simulink model "ASM_Traffic"  (R2026a)
settings: Solver=ode1  StartTime=SIM.tstart.v  StopTime=SIM.tend.v  FixedStep=SIM.StepSize.v
PostLoadFcn:
  | if any(exist('dsrtsu_mdlpostloadfcn', 'file') ~= 0), dsrtsu_mdlpostloadfcn('Execute', bdroot); end
  | try, asm_mdl_postloadfcn(bdroot, 'UpdateModel', 3600); catch, disp(lasterr); end,
InitFcn:
  | , if any(exist('rtifpga_mdlclblib', 'file') ~= 0), rtifpga_mdlclblib('Init', bdroot); end,
  | , if any(exist('dsmpb_private', 'file') ~= 0), dsmpb_private('dsmpb_mdlclblib', 'Init', bdroot); end,
model workspace (MAT data in the model file):
  asmReferencePath = [0 0.01 0.02 0.03 0.04 0.05 0.06 0.07 0.08 0.09 0.1 0.11 ... (350007 elements, 50001x7)]
  roadBounds : Simulink.Parameter (value not decoded)
  safetyAxes : Simulink.Parameter (value not decoded)
undefined symbols (not defined in the file): _to_, a0b2, ASM_BrakeHydraulics_DemoSystems, ASM_VehicleDynamics_DemoSystems, b98103fe8ad365046cd0, BrakeCircuit, controllerConfig, CPT, Crankshaft, DiscIntNeverNeededParam, dsmsi, FinalDriveAssembly, MDL, ModeSignals, mu, Pos_BrakePedal_Maneuver, rad, RefSignals, roadFamilyData, roadFamilyId, s_to_rpm, SIM, SoftECU, Suspension, Tire, Transmission
libraries: ASM_Traffic_lib x135, simulink x98, ASM_Utils_lib x77, ASM_VehicleDynamics_lib x70, ASM_Environment_lib x22, dsmpblib x20, dsmsilib x15, MDLD_Utils_lib x10, ASM_BrakeHydraulics_lib x3, sl_discontinuities x2
(part 10 of 65)

== system ASM_Traffic/AnimationInterface/Fellow_Doors/Select_Signals ==
  Fellow_Doors : Inport
  Bus Selector1 : BusSelector  OutputSignals=Settings.FellowVehicleDoors.Fellow1_Doors.SW_ManualControl_Doors[1Scheduler|2Manual],Settings.FellowVehicleDoors.Fellow2_Doors.SW_ManualControl_Doors[1Scheduler|2Manual],Settings.FellowVehicleDoors.Fellow3_Doors.SW_ManualControl_Doors[1Scheduler|2Manual],Settings.FellowVehicleDoors.Fellow4_Doors.SW_ManualControl_Doors[1Scheduler|2Manual],Settings.FellowVehicleDoors.Fellow5_Doors.SW_ManualControl_Doors[1Scheduler|2Manual],Settings.FellowVehicleDoors.Fellow6_Doors.SW_ManualControl_Doors[1Scheduler|2Manual],Settings.FellowVehicleDoors.Fellow7_Doors.SW_ManualControl_Doors[1Scheduler|2Manual],Settings.FellowVehicleDoors.Fellow8_Doors.SW_ManualControl_Doors[1Scheduler|2Manual],Settings.FellowVehicleDoors.Fellow9_Doors.SW_ManualControl_Doors[1Scheduler|2Manual],Settings.FellowVehicleDoors.Fellow10_Doors.SW_ManualControl_Doors[1Scheduler|2Manual],Settings.FellowVehicleDoors.Fellow11_Doors.SW_ManualControl_Doors[1Scheduler|2Manual],Settings.FellowVehicleDoors.Fellow12_Doors.SW_ManualControl_Doors[1Scheduler|2Manual],Settings.FellowVehicleDoors.Fellow13_Doors.SW_ManualControl_Doors[1Scheduler|2Manual],Settings.FellowVehicleDoors.Fellow14_Doors.SW_ManualControl_Doors[1Scheduler|2Manual],Settings.FellowVehicleDoors.Fellow15_Doors.SW_ManualControl_Doors[1Scheduler|2Manual],Settings.FellowVehicleDoors.Fellow16_Doors.SW_ManualControl_Doors[1Scheduler|2Manual],Settings.FellowVehicleDoors.Fellow17_Doors.SW_ManualControl_Doors[1Scheduler|2Manual],Settings.FellowVehicleDoors.Fellow18_Doors.SW_ManualControl_Doors[1Scheduler|2Manual],Settings.FellowVehicleDoors.Fellow19_Doors.SW_ManualControl_Doors[1Scheduler|2Manual],Settings.FellowVehicleDoors.Fellow20_Doors.SW_ManualControl_Doors[1Scheduler|2Manual],Settings.FellowVehicleDoors.Fellow21_Doors.SW_ManualControl_Doors[1Scheduler|2Manual],Settings.FellowVehicleDoors.Fellow22_Doors.SW_ManualControl_Doors[1Scheduler|2Manual],Settings.FellowVehicleDoors.Fellow23_Doors.SW_ManualControl_Doors[1Scheduler|2Manual],Settings.FellowVehicleDoors.Fellow24_Doors.SW_ManualControl_Doors[1Scheduler|2Manual],Settings.FellowVehicleDoors.Fellow25_Doors.SW_ManualControl_Doors[1Scheduler|2Manual],Settings.FellowVehicleDoors.Fellow26_Doors.SW_ManualControl_Doors[1Scheduler|2Manual],Settings.FellowVehicleDoors.Fellow27_Doors.SW_ManualControl_Doors[1Scheduler|2Manual],Settings.FellowVehicleDoors.Fellow28_Doors.SW_ManualControl_Doors[1Scheduler|2Manual],Settings.FellowVehicleDoors.Fellow29_Doors.SW_ManualControl_Doors[1Scheduler|2Manual],Settings.FellowVehicleDoors.Fellow30_Doors.SW_ManualControl_Doors[1Scheduler|2Manual]
  Bus Selector2 : BusSelector  OutputSignals=Settings.FellowVehicleDoors.Fellow1_Doors.SW_DoorFL[0Closed_1Open],Settings.FellowVehicleDoors.Fellow2_Doors.SW_DoorFL[0Closed_1Open],Settings.FellowVehicleDoors.Fellow3_Doors.SW_DoorFL[0Closed_1Open],Settings.FellowVehicleDoors.Fellow4_Doors.SW_DoorFL[0Closed_1Open],Settings.FellowVehicleDoors.Fellow5_Doors.SW_DoorFL[0Closed_1Open],Settings.FellowVehicleDoors.Fellow6_Doors.SW_DoorFL[0Closed_1Open],Settings.FellowVehicleDoors.Fellow7_Doors.SW_DoorFL[0Closed_1Open],Settings.FellowVehicleDoors.Fellow8_Doors.SW_DoorFL[0Closed_1Open],Settings.FellowVehicleDoors.Fellow9_Doors.SW_DoorFL[0Closed_1Open],Settings.FellowVehicleDoors.Fellow10_Doors.SW_DoorFL[0Closed_1Open],Settings.FellowVehicleDoors.Fellow11_Doors.SW_DoorFL[0Closed_1Open],Settings.FellowVehicleDoors.Fellow12_Doors.SW_DoorFL[0Closed_1Open],Settings.FellowVehicleDoors.Fellow13_Doors.SW_DoorFL[0Closed_1Open],Settings.FellowVehicleDoors.Fellow14_Doors.SW_DoorFL[0Closed_1Open],Settings.FellowVehicleDoors.Fellow15_Doors.SW_DoorFL[0Closed_1Open],Settings.FellowVehicleDoors.Fellow16_Doors.SW_DoorFL[0Closed_1Open],Settings.FellowVehicleDoors.Fellow17_Doors.SW_DoorFL[0Closed_1Open],Settings.FellowVehicleDoors.Fellow18_Doors.SW_DoorFL[0Closed_1Open],Settings.FellowVehicleDoors.Fellow19_Doors.SW_DoorFL[0Closed_1Open],Settings.FellowVehicleDoors.Fellow20_Doors.SW_DoorFL[0Closed_1Open],Settings.FellowVehicleDoors.Fellow21_Doors.SW_DoorFL[0Closed_1Open],Settings.FellowVehicleDoors.Fellow22_Doors.SW_DoorFL[0Closed_1Open],Settings.FellowVehicleDoors.Fellow23_Doors.SW_DoorFL[0Closed_1Open],Settings.FellowVehicleDoors.Fellow24_Doors.SW_DoorFL[0Closed_1Open],Settings.FellowVehicleDoors.Fellow25_Doors.SW_DoorFL[0Closed_1Open],Settings.FellowVehicleDoors.Fellow26_Doors.SW_DoorFL[0Closed_1Open],Settings.FellowVehicleDoors.Fellow27_Doors.SW_DoorFL[0Closed_1Open],Settings.FellowVehicleDoors.Fellow28_Doors.SW_DoorFL[0Closed_1Open],Settings.FellowVehicleDoors.Fellow29_Doors.SW_DoorFL[0Closed_1Open],Settings.FellowVehicleDoors.Fellow30_Doors.SW_DoorFL[0Closed_1Open]
  Bus Selector3 : BusSelector  OutputSignals=Settings.FellowVehicleDoors.Fellow1_Doors.SW_DoorFR[0Closed_1Open],Settings.FellowVehicleDoors.Fellow2_Doors.SW_DoorFR[0Closed_1Open],Settings.FellowVehicleDoors.Fellow3_Doors.SW_DoorFR[0Closed_1Open],Settings.FellowVehicleDoors.Fellow4_Doors.SW_DoorFR[0Closed_1Open],Settings.FellowVehicleDoors.Fellow5_Doors.SW_DoorFR[0Closed_1Open],Settings.FellowVehicleDoors.Fellow6_Doors.SW_DoorFR[0Closed_1Open],Settings.FellowVehicleDoors.Fellow7_Doors.SW_DoorFR[0Closed_1Open],Settings.FellowVehicleDoors.Fellow8_Doors.SW_DoorFR[0Closed_1Open],Settings.FellowVehicleDoors.Fellow9_Doors.SW_DoorFR[0Closed_1Open],Settings.FellowVehicleDoors.Fellow10_Doors.SW_DoorFR[0Closed_1Open],Settings.FellowVehicleDoors.Fellow11_Doors.SW_DoorFR[0Closed_1Open],Settings.FellowVehicleDoors.Fellow12_Doors.SW_DoorFR[0Closed_1Open],Settings.FellowVehicleDoors.Fellow13_Doors.SW_DoorFR[0Closed_1Open],Settings.FellowVehicleDoors.Fellow14_Doors.SW_DoorFR[0Closed_1Open],Settings.FellowVehicleDoors.Fellow15_Doors.SW_DoorFR[0Closed_1Open],Settings.FellowVehicleDoors.Fellow16_Doors.SW_DoorFR[0Closed_1Open],Settings.FellowVehicleDoors.Fellow17_Doors.SW_DoorFR[0Closed_1Open],Settings.FellowVehicleDoors.Fellow18_Doors.SW_DoorFR[0Closed_1Open],Settings.FellowVehicleDoors.Fellow19_Doors.SW_DoorFR[0Closed_1Open],Settings.FellowVehicleDoors.Fellow20_Doors.SW_DoorFR[0Closed_1Open],Settings.FellowVehicleDoors.Fellow21_Doors.SW_DoorFR[0Closed_1Open],Settings.FellowVehicleDoors.Fellow22_Doors.SW_DoorFR[0Closed_1Open],Settings.FellowVehicleDoors.Fellow23_Doors.SW_DoorFR[0Closed_1Open],Settings.FellowVehicleDoors.Fellow24_Doors.SW_DoorFR[0Closed_1Open],Settings.FellowVehicleDoors.Fellow25_Doors.SW_DoorFR[0Closed_1Open],Settings.FellowVehicleDoors.Fellow26_Doors.SW_DoorFR[0Closed_1Open],Settings.FellowVehicleDoors.Fellow27_Doors.SW_DoorFR[0Closed_1Open],Settings.FellowVehicleDoors.Fellow28_Doors.SW_DoorFR[0Closed_1Open],Settings.FellowVehicleDoors.Fellow29_Doors.SW_DoorFR[0Closed_1Open],Settings.FellowVehicleDoors.Fellow30_Doors.SW_DoorFR[0Closed_1Open]
  Bus Selector4 : BusSelector  OutputSignals=Settings.FellowVehicleDoors.Fellow1_Doors.SW_DoorRL[0Closed_1Open],Settings.FellowVehicleDoors.Fellow2_Doors.SW_DoorRL[0Closed_1Open],Settings.FellowVehicleDoors.Fellow3_Doors.SW_DoorRL[0Closed_1Open],Settings.FellowVehicleDoors.Fellow4_Doors.SW_DoorRL[0Closed_1Open],Settings.FellowVehicleDoors.Fellow5_Doors.SW_DoorRL[0Closed_1Open],Settings.FellowVehicleDoors.Fellow6_Doors.SW_DoorRL[0Closed_1Open],Settings.FellowVehicleDoors.Fellow7_Doors.SW_DoorRL[0Closed_1Open],Settings.FellowVehicleDoors.Fellow8_Doors.SW_DoorRL[0Closed_1Open],Settings.FellowVehicleDoors.Fellow9_Doors.SW_DoorRL[0Closed_1Open],Settings.FellowVehicleDoors.Fellow10_Doors.SW_DoorRL[0Closed_1Open],Settings.FellowVehicleDoors.Fellow11_Doors.SW_DoorRL[0Closed_1Open],Settings.FellowVehicleDoors.Fellow12_Doors.SW_DoorRL[0Closed_1Open],Settings.FellowVehicleDoors.Fellow13_Doors.SW_DoorRL[0Closed_1Open],Settings.FellowVehicleDoors.Fellow14_Doors.SW_DoorRL[0Closed_1Open],Settings.FellowVehicleDoors.Fellow15_Doors.SW_DoorRL[0Closed_1Open],Settings.FellowVehicleDoors.Fellow16_Doors.SW_DoorRL[0Closed_1Open],Settings.FellowVehicleDoors.Fellow17_Doors.SW_DoorRL[0Closed_1Open],Settings.FellowVehicleDoors.Fellow18_Doors.SW_DoorRL[0Closed_1Open],Settings.FellowVehicleDoors.Fellow19_Doors.SW_DoorRL[0Closed_1Open],Settings.FellowVehicleDoors.Fellow20_Doors.SW_DoorRL[0Closed_1Open],Settings.FellowVehicleDoors.Fellow21_Doors.SW_DoorRL[0Closed_1Open],Settings.FellowVehicleDoors.Fellow22_Doors.SW_DoorRL[0Closed_1Open],Settings.FellowVehicleDoors.Fellow23_Doors.SW_DoorRL[0Closed_1Open],Settings.FellowVehicleDoors.Fellow24_Doors.SW_DoorRL[0Closed_1Open],Settings.FellowVehicleDoors.Fellow25_Doors.SW_DoorRL[0Closed_1Open],Settings.FellowVehicleDoors.Fellow26_Doors.SW_DoorRL[0Closed_1Open],Settings.FellowVehicleDoors.Fellow27_Doors.SW_DoorRL[0Closed_1Open],Settings.FellowVehicleDoors.Fellow28_Doors.SW_DoorRL[0Closed_1Open],Settings.FellowVehicleDoors.Fellow29_Doors.SW_DoorRL[0Closed_1Open],Settings.FellowVehicleDoors.Fellow30_Doors.SW_DoorRL[0Closed_1Open]
  Bus Selector5 : BusSelector  OutputSignals=Settings.FellowVehicleDoors.Fellow1_Doors.SW_DoorRR[0Closed_1Open],Settings.FellowVehicleDoors.Fellow2_Doors.SW_DoorRR[0Closed_1Open],Settings.FellowVehicleDoors.Fellow3_Doors.SW_DoorRR[0Closed_1Open],Settings.FellowVehicleDoors.Fellow4_Doors.SW_DoorRR[0Closed_1Open],Settings.FellowVehicleDoors.Fellow5_Doors.SW_DoorRR[0Closed_1Open],Settings.FellowVehicleDoors.Fellow6_Doors.SW_DoorRR[0Closed_1Open],Settings.FellowVehicleDoors.Fellow7_Doors.SW_DoorRR[0Closed_1Open],Settings.FellowVehicleDoors.Fellow8_Doors.SW_DoorRR[0Closed_1Open],Settings.FellowVehicleDoors.Fellow9_Doors.SW_DoorRR[0Closed_1Open],Settings.FellowVehicleDoors.Fellow10_Doors.SW_DoorRR[0Closed_1Open],Settings.FellowVehicleDoors.Fellow11_Doors.SW_DoorRR[0Closed_1Open],Settings.FellowVehicleDoors.Fellow12_Doors.SW_DoorRR[0Closed_1Open],Settings.FellowVehicleDoors.Fellow13_Doors.SW_DoorRR[0Closed_1Open],Settings.FellowVehicleDoors.Fellow14_Doors.SW_DoorRR[0Closed_1Open],Settings.FellowVehicleDoors.Fellow15_Doors.SW_DoorRR[0Closed_1Open],Settings.FellowVehicleDoors.Fellow16_Doors.SW_DoorRR[0Closed_1Open],Settings.FellowVehicleDoors.Fellow17_Doors.SW_DoorRR[0Closed_1Open],Settings.FellowVehicleDoors.Fellow18_Doors.SW_DoorRR[0Closed_1Open],Settings.FellowVehicleDoors.Fellow19_Doors.SW_DoorRR[0Closed_1Open],Settings.FellowVehicleDoors.Fellow20_Doors.SW_DoorRR[0Closed_1Open],Settings.FellowVehicleDoors.Fellow21_Doors.SW_DoorRR[0Closed_1Open],Settings.FellowVehicleDoors.Fellow22_Doors.SW_DoorRR[0Closed_1Open],Settings.FellowVehicleDoors.Fellow23_Doors.SW_DoorRR[0Closed_1Open],Settings.FellowVehicleDoors.Fellow24_Doors.SW_DoorRR[0Closed_1Open],Settings.FellowVehicleDoors.Fellow25_Doors.SW_DoorRR[0Closed_1Open],Settings.FellowVehicleDoors.Fellow26_Doors.SW_DoorRR[0Closed_1Open],Settings.FellowVehicleDoors.Fellow27_Doors.SW_DoorRR[0Closed_1Open],Settings.FellowVehicleDoors.Fellow28_Doors.SW_DoorRR[0Closed_1Open],Settings.FellowVehicleDoors.Fellow29_Doors.SW_DoorRR[0Closed_1Open],Settings.FellowVehicleDoors.Fellow30_Doors.SW_DoorRR[0Closed_1Open]
  Bus Selector6 : BusSelector  OutputSignals=Settings.FellowVehicleDoors.Fellow1_Doors.SW_Hood[0Closed_1Open],Settings.FellowVehicleDoors.Fellow2_Doors.SW_Hood[0Closed_1Open],Settings.FellowVehicleDoors.Fellow3_Doors.SW_Hood[0Closed_1Open],Settings.FellowVehicleDoors.Fellow4_Doors.SW_Hood[0Closed_1Open],Settings.FellowVehicleDoors.Fellow5_Doors.SW_Hood[0Closed_1Open],Settings.FellowVehicleDoors.Fellow6_Doors.SW_Hood[0Closed_1Open],Settings.FellowVehicleDoors.Fellow7_Doors.SW_Hood[0Closed_1Open],Settings.FellowVehicleDoors.Fellow8_Doors.SW_Hood[0Closed_1Open],Settings.FellowVehicleDoors.Fellow9_Doors.SW_Hood[0Closed_1Open],Settings.FellowVehicleDoors.Fellow10_Doors.SW_Hood[0Closed_1Open],Settings.FellowVehicleDoors.Fellow11_Doors.SW_Hood[0Closed_1Open],Settings.FellowVehicleDoors.Fellow12_Doors.SW_Hood[0Closed_1Open],Settings.FellowVehicleDoors.Fellow13_Doors.SW_Hood[0Closed_1Open],Settings.FellowVehicleDoors.Fellow14_Doors.SW_Hood[0Closed_1Open],Settings.FellowVehicleDoors.Fellow15_Doors.SW_Hood[0Closed_1Open],Settings.FellowVehicleDoors.Fellow16_Doors.SW_Hood[0Closed_1Open],Settings.FellowVehicleDoors.Fellow17_Doors.SW_Hood[0Closed_1Open],Settings.FellowVehicleDoors.Fellow18_Doors.SW_Hood[0Closed_1Open],Settings.FellowVehicleDoors.Fellow19_Doors.SW_Hood[0Closed_1Open],Settings.FellowVehicleDoors.Fellow20_Doors.SW_Hood[0Closed_1Open],Settings.FellowVehicleDoors.Fellow21_Doors.SW_Hood[0Closed_1Open],Settings.FellowVehicleDoors.Fellow22_Doors.SW_Hood[0Closed_1Open],Settings.FellowVehicleDoors.Fellow23_Doors.SW_Hood[0Closed_1Open],Settings.FellowVehicleDoors.Fellow24_Doors.SW_Hood[0Closed_1Open],Settings.FellowVehicleDoors.Fellow25_Doors.SW_Hood[0Closed_1Open],Settings.FellowVehicleDoors.Fellow26_Doors.SW_Hood[0Closed_1Open],Settings.FellowVehicleDoors.Fellow27_Doors.SW_Hood[0Closed_1Open],Settings.FellowVehicleDoors.Fellow28_Doors.SW_Hood[0Closed_1Open],Settings.FellowVehicleDoors.Fellow29_Doors.SW_Hood[0Closed_1Open],Settings.FellowVehicleDoors.Fellow30_Doors.SW_Hood[0Closed_1Open]
  Bus Selector7 : BusSelector  OutputSignals=Settings.FellowVehicleDoors.Fellow1_Doors.SW_Trunk[0Closed_1Open],Settings.FellowVehicleDoors.Fellow2_Doors.SW_Trunk[0Closed_1Open],Settings.FellowVehicleDoors.Fellow3_Doors.SW_Trunk[0Closed_1Open],Settings.FellowVehicleDoors.Fellow4_Doors.SW_Trunk[0Closed_1Open],Settings.FellowVehicleDoors.Fellow5_Doors.SW_Trunk[0Closed_1Open],Settings.FellowVehicleDoors.Fellow6_Doors.SW_Trunk[0Closed_1Open],Settings.FellowVehicleDoors.Fellow7_Doors.SW_Trunk[0Closed_1Open],Settings.FellowVehicleDoors.Fellow8_Doors.SW_Trunk[0Closed_1Open],Settings.FellowVehicleDoors.Fellow9_Doors.SW_Trunk[0Closed_1Open],Settings.FellowVehicleDoors.Fellow10_Doors.SW_Trunk[0Closed_1Open],Settings.FellowVehicleDoors.Fellow11_Doors.SW_Trunk[0Closed_1Open],Settings.FellowVehicleDoors.Fellow12_Doors.SW_Trunk[0Closed_1Open],Settings.FellowVehicleDoors.Fellow13_Doors.SW_Trunk[0Closed_1Open],Settings.FellowVehicleDoors.Fellow14_Doors.SW_Trunk[0Closed_1Open],Settings.FellowVehicleDoors.Fellow15_Doors.SW_Trunk[0Closed_1Open],Settings.FellowVehicleDoors.Fellow16_Doors.SW_Trunk[0Closed_1Open],Settings.FellowVehicleDoors.Fellow17_Doors.SW_Trunk[0Closed_1Open],Settings.FellowVehicleDoors.Fellow18_Doors.SW_Trunk[0Closed_1Open],Settings.FellowVehicleDoors.Fellow19_Doors.SW_Trunk[0Closed_1Open],Settings.FellowVehicleDoors.Fellow20_Doors.SW_Trunk[0Closed_1Open],Settings.FellowVehicleDoors.Fellow21_Doors.SW_Trunk[0Closed_1Open],Settings.FellowVehicleDoors.Fellow22_Doors.SW_Trunk[0Closed_1Open],Settings.FellowVehicleDoors.Fellow23_Doors.SW_Trunk[0Closed_1Open],Settings.FellowVehicleDoors.Fellow24_Doors.SW_Trunk[0Closed_1Open],Settings.FellowVehicleDoors.Fellow25_Doors.SW_Trunk[0Closed_1Open],Settings.FellowVehicleDoors.Fellow26_Doors.SW_Trunk[0Closed_1Open],Settings.FellowVehicleDoors.Fellow27_Doors.SW_Trunk[0Closed_1Open],Settings.FellowVehicleDoors.Fellow28_Doors.SW_Trunk[0Closed_1Open],Settings.FellowVehicleDoors.Fellow29_Doors.SW_Trunk[0Closed_1Open],Settings.FellowVehicleDoors.Fellow30_Doors.SW_Trunk[0Closed_1Open]
  Cast_to_boolean{,1..5} (6 alike) : DataTypeConversion  OutDataTypeStr=double  SaturateOnIntegerOverflow=off  RndMeth=Floor
  Cast_to_uint32 : DataTypeConversion  OutDataTypeStr=uint32  SaturateOnIntegerOverflow=off  RndMeth=Floor
  Mux{,1..6} (7 alike) : Mux  Inputs=30
  SW_ManualControl_Doors[1Scheduler|2Manual] : Outport
  SW_DoorFL[Open0_1Closed] : Outport  Port=2
  SW_DoorFR[Open0_1Closed] : Outport  Port=3
  SW_DoorRL[Open0_1Closed] : Outport  Port=4
  SW_DoorRR[Open0_1Closed] : Outport  Port=5
  SW_Hood[Open0_1Closed] : Outport  Port=6
  SW_Trunk[Open0_1Closed] : Outport  Port=7
  wires:
  Bus Selector1/30 -> Mux/30  "<SW_ManualControl_Doors[1Scheduler|2Manual]>"
  Bus Selector1/29 -> Mux/29  "<SW_ManualControl_Doors[1Scheduler|2Manual]>"
  Bus Selector1/28 -> Mux/28  "<SW_ManualControl_Doors[1Scheduler|2Manual]>"
  Bus Selector1/27 -> Mux/27  "<SW_ManualControl_Doors[1Scheduler|2Manual]>"
  Bus Selector1/26 -> Mux/26  "<SW_ManualControl_Doors[1Scheduler|2Manual]>"
  Bus Selector1/25 -> Mux/25  "<SW_ManualControl_Doors[1Scheduler|2Manual]>"
  Bus Selector1/24 -> Mux/24  "<SW_ManualControl_Doors[1Scheduler|2Manual]>"
  Bus Selector1/23 -> Mux/23  "<SW_ManualControl_Doors[1Scheduler|2Manual]>"
  Bus Selector1/22 -> Mux/22  "<SW_ManualControl_Doors[1Scheduler|2Manual]>"
  Bus Selector1/21 -> Mux/21  "<SW_ManualControl_Doors[1Scheduler|2Manual]>"
  Bus Selector1/20 -> Mux/20  "<SW_ManualControl_Doors[1Scheduler|2Manual]>"
  Bus Selector1/19 -> Mux/19  "<SW_ManualControl_Doors[1Scheduler|2Manual]>"
  Bus Selector1/18 -> Mux/18  "<SW_ManualControl_Doors[1Scheduler|2Manual]>"
  Bus Selector1/17 -> Mux/17  "<SW_ManualControl_Doors[1Scheduler|2Manual]>"
  Bus Selector1/16 -> Mux/16  "<SW_ManualControl_Doors[1Scheduler|2Manual]>"
  Bus Selector1/15 -> Mux/15  "<SW_ManualControl_Doors[1Scheduler|2Manual]>"
  Bus Selector1/14 -> Mux/14  "<SW_ManualControl_Doors[1Scheduler|2Manual]>"
  Bus Selector1/13 -> Mux/13  "<SW_ManualControl_Doors[1Scheduler|2Manual]>"
  Bus Selector1/12 -> Mux/12  "<SW_ManualControl_Doors[1Scheduler|2Manual]>"
  Bus Selector1/11 -> Mux/11  "<SW_ManualControl_Doors[1Scheduler|2Manual]>"
  Bus Selector1/10 -> Mux/10  "<SW_ManualControl_Doors[1Scheduler|2Manual]>"
  Bus Selector1/9 -> Mux/9  "<SW_ManualControl_Doors[1Scheduler|2Manual]>"
  Bus Selector1/8 -> Mux/8  "<SW_ManualControl_Doors[1Scheduler|2Manual]>"
  Bus Selector1/7 -> Mux/7  "<SW_ManualControl_Doors[1Scheduler|2Manual]>"
  Bus Selector1/6 -> Mux/6  "<SW_ManualControl_Doors[1Scheduler|2Manual]>"
  Bus Selector1/5 -> Mux/5  "<SW_ManualControl_Doors[1Scheduler|2Manual]>"
  Bus Selector1/4 -> Mux/4  "<SW_ManualControl_Doors[1Scheduler|2Manual]>"
  Bus Selector1/3 -> Mux/3  "<SW_ManualControl_Doors[1Scheduler|2Manual]>"
  Bus Selector1/2 -> Mux/2  "<SW_ManualControl_Doors[1Scheduler|2Manual]>"
  Bus Selector1/1 -> Mux/1  "<SW_ManualControl_Doors[1Scheduler|2Manual]>"
  Bus Selector7/15 -> Mux6/15  "<SW_Trunk[0Closed_1Open]>"
  Bus Selector7/7 -> Mux6/7  "<SW_Trunk[0Closed_1Open]>"
  Bus Selector7/12 -> Mux6/12  "<SW_Trunk[0Closed_1Open]>"
  Bus Selector7/1 -> Mux6/1  "<SW_Trunk[0Closed_1Open]>"
  Bus Selector7/18 -> Mux6/18  "<SW_Trunk[0Closed_1Open]>"
  Bus Selector7/28 -> Mux6/28  "<SW_Trunk[0Closed_1Open]>"
  Bus Selector7/5 -> Mux6/5  "<SW_Trunk[0Closed_1Open]>"
  Bus Selector7/27 -> Mux6/27  "<SW_Trunk[0Closed_1Open]>"
  Bus Selector7/26 -> Mux6/26  "<SW_Trunk[0Closed_1Open]>"
  Bus Selector7/6 -> Mux6/6  "<SW_Trunk[0Closed_1Open]>"
  Bus Selector7/21 -> Mux6/21  "<SW_Trunk[0Closed_1Open]>"
  Bus Selector7/17 -> Mux6/17  "<SW_Trunk[0Closed_1Open]>"
  Bus Selector7/25 -> Mux6/25  "<SW_Trunk[0Closed_1Open]>"
  Cast_to_boolean5/1 -> SW_Trunk[Open0_1Closed]/1
  Bus Selector7/9 -> Mux6/9  "<SW_Trunk[0Closed_1Open]>"
  Fellow_Doors/1 -> Bus Selector1/1, Bus Selector2/1, Bus Selector3/1, Bus Selector4/1, Bus Selector5/1, Bus Selector6/1, Bus Selector7/1
  Bus Selector7/10 -> Mux6/10  "<SW_Trunk[0Closed_1Open]>"
  Bus Selector7/4 -> Mux6/4  "<SW_Trunk[0Closed_1Open]>"
  Bus Selector7/2 -> Mux6/2  "<SW_Trunk[0Closed_1Open]>"
  Bus Selector7/14 -> Mux6/14  "<SW_Trunk[0Closed_1Open]>"
  Bus Selector7/16 -> Mux6/16  "<SW_Trunk[0Closed_1Open]>"
  Bus Selector7/11 -> Mux6/11  "<SW_Trunk[0Closed_1Open]>"
  Bus Selector7/30 -> Mux6/30  "<SW_Trunk[0Closed_1Open]>"
  Mux6/1 -> Cast_to_boolean5/1
  Bus Selector7/19 -> Mux6/19  "<SW_Trunk[0Closed_1Open]>"
  Bus Selector7/13 -> Mux6/13  "<SW_Trunk[0Closed_1Open]>"
  Bus Selector7/20 -> Mux6/20  "<SW_Trunk[0Closed_1Open]>"
  Bus Selector7/3 -> Mux6/3  "<SW_Trunk[0Closed_1Open]>"
  Bus Selector7/22 -> Mux6/22  "<SW_Trunk[0Closed_1Open]>"
  Bus Selector7/23 -> Mux6/23  "<SW_Trunk[0Closed_1Open]>"
  Bus Selector7/24 -> Mux6/24  "<SW_Trunk[0Closed_1Open]>"
  Bus Selector7/8 -> Mux6/8  "<SW_Trunk[0Closed_1Open]>"
  Bus Selector7/29 -> Mux6/29  "<SW_Trunk[0Closed_1Open]>"
  Bus Selector6/15 -> Mux5/15  "<SW_Hood[0Closed_1Open]>"
  Bus Selector6/7 -> Mux5/7  "<SW_Hood[0Closed_1Open]>"
  Bus Selector6/12 -> Mux5/12  "<SW_Hood[0Closed_1Open]>"
  Bus Selector6/1 -> Mux5/1  "<SW_Hood[0Closed_1Open]>"
  Bus Selector6/18 -> Mux5/18  "<SW_Hood[0Closed_1Open]>"
  Bus Selector6/28 -> Mux5/28  "<SW_Hood[0Closed_1Open]>"
  Bus Selector6/5 -> Mux5/5  "<SW_Hood[0Closed_1Open]>"
  Bus Selector6/27 -> Mux5/27  "<SW_Hood[0Closed_1Open]>"
  Bus Selector6/26 -> Mux5/26  "<SW_Hood[0Closed_1Open]>"
  Bus Selector6/6 -> Mux5/6  "<SW_Hood[0Closed_1Open]>"
  Bus Selector6/21 -> Mux5/21  "<SW_Hood[0Closed_1Open]>"
  Bus Selector6/17 -> Mux5/17  "<SW_Hood[0Closed_1Open]>"
  Bus Selector6/25 -> Mux5/25  "<SW_Hood[0Closed_1Open]>"
  Cast_to_boolean4/1 -> SW_Hood[Open0_1Closed]/1
  Bus Selector6/9 -> Mux5/9  "<SW_Hood[0Closed_1Open]>"
  Bus Selector6/10 -> Mux5/10  "<SW_Hood[0Closed_1Open]>"
  Bus Selector6/4 -> Mux5/4  "<SW_Hood[0Closed_1Open]>"
  Bus Selector6/2 -> Mux5/2  "<SW_Hood[0Closed_1Open]>"
  Bus Selector6/14 -> Mux5/14  "<SW_Hood[0Closed_1Open]>"
  Bus Selector6/16 -> Mux5/16  "<SW_Hood[0Closed_1Open]>"
  Bus Selector6/11 -> Mux5/11  "<SW_Hood[0Closed_1Open]>"
  Bus Selector6/30 -> Mux5/30  "<SW_Hood[0Closed_1Open]>"
  Mux5/1 -> Cast_to_boolean4/1
  Bus Selector6/19 -> Mux5/19  "<SW_Hood[0Closed_1Open]>"
  Bus Selector6/13 -> Mux5/13  "<SW_Hood[0Closed_1Open]>"
  Bus Selector6/20 -> Mux5/20  "<SW_Hood[0Closed_1Open]>"
  Bus Selector6/3 -> Mux5/3  "<SW_Hood[0Closed_1Open]>"
  Bus Selector6/22 -> Mux5/22  "<SW_Hood[0Closed_1Open]>"
  Bus Selector6/23 -> Mux5/23  "<SW_Hood[0Closed_1Open]>"
  Bus Selector6/24 -> Mux5/24  "<SW_Hood[0Closed_1Open]>"
  Bus Selector6/8 -> Mux5/8  "<SW_Hood[0Closed_1Open]>"
  Bus Selector6/29 -> Mux5/29  "<SW_Hood[0Closed_1Open]>"
  Bus Selector5/15 -> Mux4/15  "<SW_DoorRR[0Closed_1Open]>"
  Bus Selector5/7 -> Mux4/7  "<SW_DoorRR[0Closed_1Open]>"
  Bus Selector5/12 -> Mux4/12  "<SW_DoorRR[0Closed_1Open]>"
  Bus Selector5/1 -> Mux4/1  "<SW_DoorRR[0Closed_1Open]>"
  Bus Selector5/18 -> Mux4/18  "<SW_DoorRR[0Closed_1Open]>"
  Bus Selector5/28 -> Mux4/28  "<SW_DoorRR[0Closed_1Open]>"
  Bus Selector5/5 -> Mux4/5  "<SW_DoorRR[0Closed_1Open]>"
  Bus Selector5/27 -> Mux4/27  "<SW_DoorRR[0Closed_1Open]>"
  Bus Selector5/26 -> Mux4/26  "<SW_DoorRR[0Closed_1Open]>"
  Bus Selector5/6 -> Mux4/6  "<SW_DoorRR[0Closed_1Open]>"
  Bus Selector5/21 -> Mux4/21  "<SW_DoorRR[0Closed_1Open]>"
  Bus Selector5/17 -> Mux4/17  "<SW_DoorRR[0Closed_1Open]>"
  Bus Selector5/25 -> Mux4/25  "<SW_DoorRR[0Closed_1Open]>"
  Cast_to_boolean3/1 -> SW_DoorRR[Open0_1Closed]/1
  Bus Selector5/9 -> Mux4/9  "<SW_DoorRR[0Closed_1Open]>"
  Bus Selector5/10 -> Mux4/10  "<SW_DoorRR[0Closed_1Open]>"
  Bus Selector5/4 -> Mux4/4  "<SW_DoorRR[0Closed_1Open]>"
  Bus Selector5/2 -> Mux4/2  "<SW_DoorRR[0Closed_1Open]>"
  Bus Selector5/14 -> Mux4/14  "<SW_DoorRR[0Closed_1Open]>"
  Bus Selector5/16 -> Mux4/16  "<SW_DoorRR[0Closed_1Open]>"
  Bus Selector5/11 -> Mux4/11  "<SW_DoorRR[0Closed_1Open]>"
  Bus Selector5/30 -> Mux4/30  "<SW_DoorRR[0Closed_1Open]>"
  Mux4/1 -> Cast_to_boolean3/1
  Bus Selector5/19 -> Mux4/19  "<SW_DoorRR[0Closed_1Open]>"
  Bus Selector5/13 -> Mux4/13  "<SW_DoorRR[0Closed_1Open]>"
  Bus Selector5/20 -> Mux4/20  "<SW_DoorRR[0Closed_1Open]>"
  Bus Selector5/3 -> Mux4/3  "<SW_DoorRR[0Closed_1Open]>"
  Bus Selector5/22 -> Mux4/22  "<SW_DoorRR[0Closed_1Open]>"
  Bus Selector5/23 -> Mux4/23  "<SW_DoorRR[0Closed_1Open]>"
  Bus Selector5/24 -> Mux4/24  "<SW_DoorRR[0Closed_1Open]>"
  Bus Selector5/8 -> Mux4/8  "<SW_DoorRR[0Closed_1Open]>"
  Bus Selector5/29 -> Mux4/29  "<SW_DoorRR[0Closed_1Open]>"
  Bus Selector4/15 -> Mux3/15  "<SW_DoorRL[0Closed_1Open]>"
  Bus Selector4/7 -> Mux3/7  "<SW_DoorRL[0Closed_1Open]>"
  Bus Selector4/12 -> Mux3/12  "<SW_DoorRL[0Closed_1Open]>"
  Bus Selector4/1 -> Mux3/1  "<SW_DoorRL[0Closed_1Open]>"
  Bus Selector4/18 -> Mux3/18  "<SW_DoorRL[0Closed_1Open]>"
  Bus Selector4/28 -> Mux3/28  "<SW_DoorRL[0Closed_1Open]>"
  Bus Selector4/5 -> Mux3/5  "<SW_DoorRL[0Closed_1Open]>"
  Bus Selector4/27 -> Mux3/27  "<SW_DoorRL[0Closed_1Open]>"
  Bus Selector4/26 -> Mux3/26  "<SW_DoorRL[0Closed_1Open]>"
  Bus Selector4/6 -> Mux3/6  "<SW_DoorRL[0Closed_1Open]>"
  Bus Selector4/21 -> Mux3/21  "<SW_DoorRL[0Closed_1Open]>"
  Bus Selector4/17 -> Mux3/17  "<SW_DoorRL[0Closed_1Open]>"
  Bus Selector4/25 -> Mux3/25  "<SW_DoorRL[0Closed_1Open]>"
  Cast_to_boolean2/1 -> SW_DoorRL[Open0_1Closed]/1
  Bus Selector4/9 -> Mux3/9  "<SW_DoorRL[0Closed_1Open]>"
  Bus Selector4/10 -> Mux3/10  "<SW_DoorRL[0Closed_1Open]>"
  Bus Selector4/4 -> Mux3/4  "<SW_DoorRL[0Closed_1Open]>"
  Bus Selector4/2 -> Mux3/2  "<SW_DoorRL[0Closed_1Open]>"
  Bus Selector4/14 -> Mux3/14  "<SW_DoorRL[0Closed_1Open]>"
  Bus Selector4/16 -> Mux3/16  "<SW_DoorRL[0Closed_1Open]>"
  Bus Selector4/11 -> Mux3/11  "<SW_DoorRL[0Closed_1Open]>"
  Bus Selector4/30 -> Mux3/30  "<SW_DoorRL[0Closed_1Open]>"
  Mux3/1 -> Cast_to_boolean2/1
  Bus Selector4/19 -> Mux3/19  "<SW_DoorRL[0Closed_1Open]>"
  Bus Selector4/13 -> Mux3/13  "<SW_DoorRL[0Closed_1Open]>"
  Bus Selector4/20 -> Mux3/20  "<SW_DoorRL[0Closed_1Open]>"
  Bus Selector4/3 -> Mux3/3  "<SW_DoorRL[0Closed_1Open]>"
  Bus Selector4/22 -> Mux3/22  "<SW_DoorRL[0Closed_1Open]>"
  Bus Selector4/23 -> Mux3/23  "<SW_DoorRL[0Closed_1Open]>"
  Bus Selector4/24 -> Mux3/24  "<SW_DoorRL[0Closed_1Open]>"
  Bus Selector4/8 -> Mux3/8  "<SW_DoorRL[0Closed_1Open]>"
  Bus Selector4/29 -> Mux3/29  "<SW_DoorRL[0Closed_1Open]>"
  Bus Selector3/15 -> Mux2/15  "<SW_DoorFR[0Closed_1Open]>"
  Bus Selector3/7 -> Mux2/7  "<SW_DoorFR[0Closed_1Open]>"
  Bus Selector3/12 -> Mux2/12  "<SW_DoorFR[0Closed_1Open]>"
  Bus Selector3/1 -> Mux2/1  "<SW_DoorFR[0Closed_1Open]>"
  Bus Selector3/18 -> Mux2/18  "<SW_DoorFR[0Closed_1Open]>"
  Bus Selector3/28 -> Mux2/28  "<SW_DoorFR[0Closed_1Open]>"
  Bus Selector3/5 -> Mux2/5  "<SW_DoorFR[0Closed_1Open]>"
  Bus Selector3/27 -> Mux2/27  "<SW_DoorFR[0Closed_1Open]>"
  Bus Selector3/26 -> Mux2/26  "<SW_DoorFR[0Closed_1Open]>"
  Bus Selector3/6 -> Mux2/6  "<SW_DoorFR[0Closed_1Open]>"
  Bus Selector3/21 -> Mux2/21  "<SW_DoorFR[0Closed_1Open]>"
  Bus Selector3/17 -> Mux2/17  "<SW_DoorFR[0Closed_1Open]>"
  Bus Selector3/25 -> Mux2/25  "<SW_DoorFR[0Closed_1Open]>"
  Cast_to_boolean1/1 -> SW_DoorFR[Open0_1Closed]/1
  Bus Selector3/9 -> Mux2/9  "<SW_DoorFR[0Closed_1Open]>"
  Bus Selector3/10 -> Mux2/10  "<SW_DoorFR[0Closed_1Open]>"
  Bus Selector3/4 -> Mux2/4  "<SW_DoorFR[0Closed_1Open]>"
  Bus Selector3/2 -> Mux2/2  "<SW_DoorFR[0Closed_1Open]>"
  Bus Selector3/14 -> Mux2/14  "<SW_DoorFR[0Closed_1Open]>"
  Bus Selector3/16 -> Mux2/16  "<SW_DoorFR[0Closed_1Open]>"
  Bus Selector3/11 -> Mux2/11  "<SW_DoorFR[0Closed_1Open]>"
  Bus Selector3/30 -> Mux2/30  "<SW_DoorFR[0Closed_1Open]>"
  Mux2/1 -> Cast_to_boolean1/1
  Bus Selector3/19 -> Mux2/19  "<SW_DoorFR[0Closed_1Open]>"
  Bus Selector3/13 -> Mux2/13  "<SW_DoorFR[0Closed_1Open]>"
  Bus Selector3/20 -> Mux2/20  "<SW_DoorFR[0Closed_1Open]>"
  Bus Selector3/3 -> Mux2/3  "<SW_DoorFR[0Closed_1Open]>"
  Bus Selector3/22 -> Mux2/22  "<SW_DoorFR[0Closed_1Open]>"
  Bus Selector3/23 -> Mux2/23  "<SW_DoorFR[0Closed_1Open]>"
  Bus Selector3/24 -> Mux2/24  "<SW_DoorFR[0Closed_1Open]>"
  Bus Selector3/8 -> Mux2/8  "<SW_DoorFR[0Closed_1Open]>"
  Bus Selector3/29 -> Mux2/29  "<SW_DoorFR[0Closed_1Open]>"
  Bus Selector2/30 -> Mux1/30  "<SW_DoorFL[0Closed_1Open]>"
  Bus Selector2/29 -> Mux1/29  "<SW_DoorFL[0Closed_1Open]>"
  Bus Selector2/28 -> Mux1/28  "<SW_DoorFL[0Closed_1Open]>"
  Bus Selector2/27 -> Mux1/27  "<SW_DoorFL[0Closed_1Open]>"
  Bus Selector2/26 -> Mux1/26  "<SW_DoorFL[0Closed_1Open]>"
  Bus Selector2/25 -> Mux1/25  "<SW_DoorFL[0Closed_1Open]>"
  Bus Selector2/24 -> Mux1/24  "<SW_DoorFL[0Closed_1Open]>"
  Bus Selector2/23 -> Mux1/23  "<SW_DoorFL[0Closed_1Open]>"
  Bus Selector2/22 -> Mux1/22  "<SW_DoorFL[0Closed_1Open]>"
  Bus Selector2/21 -> Mux1/21  "<SW_DoorFL[0Closed_1Open]>"
  Bus Selector2/20 -> Mux1/20  "<SW_DoorFL[0Closed_1Open]>"
  Bus Selector2/19 -> Mux1/19  "<SW_DoorFL[0Closed_1Open]>"
  Bus Selector2/18 -> Mux1/18  "<SW_DoorFL[0Closed_1Open]>"
  Bus Selector2/17 -> Mux1/17  "<SW_DoorFL[0Closed_1Open]>"
  Bus Selector2/16 -> Mux1/16  "<SW_DoorFL[0Closed_1Open]>"
  Bus Selector2/15 -> Mux1/15  "<SW_DoorFL[0Closed_1Open]>"
  Bus Selector2/14 -> Mux1/14  "<SW_DoorFL[0Closed_1Open]>"
  Bus Selector2/13 -> Mux1/13  "<SW_DoorFL[0Closed_1Open]>"
  Bus Selector2/12 -> Mux1/12  "<SW_DoorFL[0Closed_1Open]>"
  Bus Selector2/11 -> Mux1/11  "<SW_DoorFL[0Closed_1Open]>"
  Bus Selector2/10 -> Mux1/10  "<SW_DoorFL[0Closed_1Open]>"
  Bus Selector2/9 -> Mux1/9  "<SW_DoorFL[0Closed_1Open]>"
  Bus Selector2/8 -> Mux1/8  "<SW_DoorFL[0Closed_1Open]>"
  Bus Selector2/7 -> Mux1/7  "<SW_DoorFL[0Closed_1Open]>"
  Bus Selector2/6 -> Mux1/6  "<SW_DoorFL[0Closed_1Open]>"
  Bus Selector2/5 -> Mux1/5  "<SW_DoorFL[0Closed_1Open]>"
  Bus Selector2/4 -> Mux1/4  "<SW_DoorFL[0Closed_1Open]>"
  Bus Selector2/3 -> Mux1/3  "<SW_DoorFL[0Closed_1Open]>"
  Bus Selector2/2 -> Mux1/2  "<SW_DoorFL[0Closed_1Open]>"
  Bus Selector2/1 -> Mux1/1  "<SW_DoorFL[0Closed_1Open]>"
  Mux1/1 -> Cast_to_boolean/1
  Mux/1 -> Cast_to_uint32/1
  Cast_to_boolean/1 -> SW_DoorFL[Open0_1Closed]/1
  Cast_to_uint32/1 -> SW_ManualControl_Doors[1Scheduler|2Manual]/1

== system ASM_Traffic/AnimationInterface/Fellow_Lights/Coding ==
  FellowLights : Inport
  BitwiseOR : simulink/Logic and Bit Operations/Bitwise Operator  logicop=OR  UseBitMask=off  NumInputPorts=3  BitMask=bin2dec('11011001')  BitMaskRealWorld=Stored Integer
  Data Type Conversion : DataTypeConversion  OutDataTypeStr=uint32  SaturateOnIntegerOverflow=off  RndMeth=Floor
  Data Type Conversion1 : DataTypeConversion  OutDataTypeStr=uint32  SaturateOnIntegerOverflow=off  RndMeth=Floor
  Demux : Demux  Outputs=3
  Gain : Gain  Gain=15  ParamDataTypeStr=uint32  OutDataTypeStr=uint32
  Gain1 : Gain  Gain=15  ParamDataTypeStr=uint32  OutDataTypeStr=uint32
  Gain2 : Gain  Gain=15  ParamDataTypeStr=uint32  OutDataTypeStr=uint32
  Shift Arithmetic : ArithShift  BitShiftNumber=4  BitShiftDirection=Left
  Shift Arithmetic1 : ArithShift  BitShiftNumber=8  BitShiftDirection=Left
  SwitchDelay : Subsystem
  Out : Outport  VectorParamsAs1DForOutWhenUnconnected=off
  wires:
  BitwiseOR/1 -> Data Type Conversion1/1
  Shift Arithmetic1/1 -> BitwiseOR/3
  FellowLights/1 -> Data Type Conversion/1
  Demux/3 -> SwitchDelay/2(Turnlight_R)
  SwitchDelay/1(Turnlight_L_out) -> Gain1/1
  Demux/2 -> SwitchDelay/1(Turnlight_L)
  Gain/1 -> BitwiseOR/1
  Demux/1 -> Gain/1
  Gain1/1 -> Shift Arithmetic/1
  Gain2/1 -> Shift Arithmetic1/1
  SwitchDelay/2(Turnlight_R_out) -> Gain2/1
  Data Type Conversion/1 -> Demux/1
  Data Type Conversion1/1 -> Out/1
  Shift Arithmetic/1 -> BitwiseOR/2

== system ASM_Traffic/AnimationInterface/Fellow_Lights/Select_Signals ==
  Fellow_VehicleLights : Inport
  Bus Selector1 : BusSelector  OutputSignals=FellowVehicleLights.Fellow1_VehicleLights.SW_ManualControl_Lights[1Scheduler|2Manual],FellowVehicleLights.Fellow2_VehicleLights.SW_ManualControl_Lights[1Scheduler|2Manual],FellowVehicleLights.Fellow3_VehicleLights.SW_ManualControl_Lights[1Scheduler|2Manual],FellowVehicleLights.Fellow4_VehicleLights.SW_ManualControl_Lights[1Scheduler|2Manual],FellowVehicleLights.Fellow5_VehicleLights.SW_ManualControl_Lights[1Scheduler|2Manual],FellowVehicleLights.Fellow6_VehicleLights.SW_ManualControl_Lights[1Scheduler|2Manual],FellowVehicleLights.Fellow7_VehicleLights.SW_ManualControl_Lights[1Scheduler|2Manual],FellowVehicleLights.Fellow8_VehicleLights.SW_ManualControl_Lights[1Scheduler|2Manual],FellowVehicleLights.Fellow9_VehicleLights.SW_ManualControl_Lights[1Scheduler|2Manual],FellowVehicleLights.Fellow10_VehicleLights.SW_ManualControl_Lights[1Scheduler|2Manual],FellowVehicleLights.Fellow11_VehicleLights.SW_ManualControl_Lights[1Scheduler|2Manual],FellowVehicleLights.Fellow12_VehicleLights.SW_ManualControl_Lights[1Scheduler|2Manual],FellowVehicleLights.Fellow13_VehicleLights.SW_ManualControl_Lights[1Scheduler|2Manual],FellowVehicleLights.Fellow14_VehicleLights.SW_ManualControl_Lights[1Scheduler|2Manual],FellowVehicleLights.Fellow15_VehicleLights.SW_ManualControl_Lights[1Scheduler|2Manual],FellowVehicleLights.Fellow16_VehicleLights.SW_ManualControl_Lights[1Scheduler|2Manual],FellowVehicleLights.Fellow17_VehicleLights.SW_ManualControl_Lights[1Scheduler|2Manual],FellowVehicleLights.Fellow18_VehicleLights.SW_ManualControl_Lights[1Scheduler|2Manual],FellowVehicleLights.Fellow19_VehicleLights.SW_ManualControl_Lights[1Scheduler|2Manual],FellowVehicleLights.Fellow20_VehicleLights.SW_ManualControl_Lights[1Scheduler|2Manual],FellowVehicleLights.Fellow21_VehicleLights.SW_ManualControl_Lights[1Scheduler|2Manual],FellowVehicleLights.Fellow22_VehicleLights.SW_ManualControl_Lights[1Scheduler|2Manual],FellowVehicleLights.Fellow23_VehicleLights.SW_ManualControl_Lights[1Scheduler|2Manual],FellowVehicleLights.Fellow24_VehicleLights.SW_ManualControl_Lights[1Scheduler|2Manual],FellowVehicleLights.Fellow25_VehicleLights.SW_ManualControl_Lights[1Scheduler|2Manual],FellowVehicleLights.Fellow26_VehicleLights.SW_ManualControl_Lights[1Scheduler|2Manual],FellowVehicleLights.Fellow27_VehicleLights.SW_ManualControl_Lights[1Scheduler|2Manual],FellowVehicleLights.Fellow28_VehicleLights.SW_ManualControl_Lights[1Scheduler|2Manual],FellowVehicleLights.Fellow29_VehicleLights.SW_ManualControl_Lights[1Scheduler|2Manual],FellowVehicleLights.Fellow30_VehicleLights.SW_ManualControl_Lights[1Scheduler|2Manual]
  Bus Selector2 : BusSelector  OutputSignals=FellowVehicleLights.Fellow1_VehicleLights.SW_BrakeLight[0Off|1On],FellowVehicleLights.Fellow2_VehicleLights.SW_BrakeLight[0Off|1On],FellowVehicleLights.Fellow3_VehicleLights.SW_BrakeLight[0Off|1On],FellowVehicleLights.Fellow4_VehicleLights.SW_BrakeLight[0Off|1On],FellowVehicleLights.Fellow5_VehicleLights.SW_BrakeLight[0Off|1On],FellowVehicleLights.Fellow6_VehicleLights.SW_BrakeLight[0Off|1On],FellowVehicleLights.Fellow7_VehicleLights.SW_BrakeLight[0Off|1On],FellowVehicleLights.Fellow8_VehicleLights.SW_BrakeLight[0Off|1On],FellowVehicleLights.Fellow9_VehicleLights.SW_BrakeLight[0Off|1On],FellowVehicleLights.Fellow10_VehicleLights.SW_BrakeLight[0Off|1On],FellowVehicleLights.Fellow11_VehicleLights.SW_BrakeLight[0Off|1On],FellowVehicleLights.Fellow12_VehicleLights.SW_BrakeLight[0Off|1On],FellowVehicleLights.Fellow13_VehicleLights.SW_BrakeLight[0Off|1On],FellowVehicleLights.Fellow14_VehicleLights.SW_BrakeLight[0Off|1On],FellowVehicleLights.Fellow15_VehicleLights.SW_BrakeLight[0Off|1On],FellowVehicleLights.Fellow16_VehicleLights.SW_BrakeLight[0Off|1On],FellowVehicleLights.Fellow17_VehicleLights.SW_BrakeLight[0Off|1On],FellowVehicleLights.Fellow18_VehicleLights.SW_BrakeLight[0Off|1On],FellowVehicleLights.Fellow19_VehicleLights.SW_BrakeLight[0Off|1On],FellowVehicleLights.Fellow20_VehicleLights.SW_BrakeLight[0Off|1On],FellowVehicleLights.Fellow21_VehicleLights.SW_BrakeLight[0Off|1On],FellowVehicleLights.Fellow22_VehicleLights.SW_BrakeLight[0Off|1On],FellowVehicleLights.Fellow23_VehicleLights.SW_BrakeLight[0Off|1On],FellowVehicleLights.Fellow24_VehicleLights.SW_BrakeLight[0Off|1On],FellowVehicleLights.Fellow25_VehicleLights.SW_BrakeLight[0Off|1On],FellowVehicleLights.Fellow26_VehicleLights.SW_BrakeLight[0Off|1On],FellowVehicleLights.Fellow27_VehicleLights.SW_BrakeLight[0Off|1On],FellowVehicleLights.Fellow28_VehicleLights.SW_BrakeLight[0Off|1On],FellowVehicleLights.Fellow29_VehicleLights.SW_BrakeLight[0Off|1On],FellowVehicleLights.Fellow30_VehicleLights.SW_BrakeLight[0Off|1On]
  Bus Selector3 : BusSelector  OutputSignals=FellowVehicleLights.Fellow1_VehicleLights.SW_TurnLights[0Off|1Left|2Right|3Both],FellowVehicleLights.Fellow2_VehicleLights.SW_TurnLights[0Off|1Left|2Right|3Both],FellowVehicleLights.Fellow3_VehicleLights.SW_TurnLights[0Off|1Left|2Right|3Both],FellowVehicleLights.Fellow4_VehicleLights.SW_TurnLights[0Off|1Left|2Right|3Both],FellowVehicleLights.Fellow5_VehicleLights.SW_TurnLights[0Off|1Left|2Right|3Both],FellowVehicleLights.Fellow6_VehicleLights.SW_TurnLights[0Off|1Left|2Right|3Both],FellowVehicleLights.Fellow7_VehicleLights.SW_TurnLights[0Off|1Left|2Right|3Both],FellowVehicleLights.Fellow8_VehicleLights.SW_TurnLights[0Off|1Left|2Right|3Both],FellowVehicleLights.Fellow9_VehicleLights.SW_TurnLights[0Off|1Left|2Right|3Both],FellowVehicleLights.Fellow10_VehicleLights.SW_TurnLights[0Off|1Left|2Right|3Both],FellowVehicleLights.Fellow11_VehicleLights.SW_TurnLights[0Off|1Left|2Right|3Both],FellowVehicleLights.Fellow12_VehicleLights.SW_TurnLights[0Off|1Left|2Right|3Both],FellowVehicleLights.Fellow13_VehicleLights.SW_TurnLights[0Off|1Left|2Right|3Both],FellowVehicleLights.Fellow14_VehicleLights.SW_TurnLights[0Off|1Left|2Right|3Both],FellowVehicleLights.Fellow15_VehicleLights.SW_TurnLights[0Off|1Left|2Right|3Both],FellowVehicleLights.Fellow16_VehicleLights.SW_TurnLights[0Off|1Left|2Right|3Both],FellowVehicleLights.Fellow17_VehicleLights.SW_TurnLights[0Off|1Left|2Right|3Both],FellowVehicleLights.Fellow18_VehicleLights.SW_TurnLights[0Off|1Left|2Right|3Both],FellowVehicleLights.Fellow19_VehicleLights.SW_TurnLights[0Off|1Left|2Right|3Both],FellowVehicleLights.Fellow20_VehicleLights.SW_TurnLights[0Off|1Left|2Right|3Both],FellowVehicleLights.Fellow21_VehicleLights.SW_TurnLights[0Off|1Left|2Right|3Both],FellowVehicleLights.Fellow22_VehicleLights.SW_TurnLights[0Off|1Left|2Right|3Both],FellowVehicleLights.Fellow23_VehicleLights.SW_TurnLights[0Off|1Left|2Right|3Both],FellowVehicleLights.Fellow24_VehicleLights.SW_TurnLights[0Off|1Left|2Right|3Both],FellowVehicleLights.Fellow25_VehicleLights.SW_TurnLights[0Off|1Left|2Right|3Both],FellowVehicleLights.Fellow26_VehicleLights.SW_TurnLights[0Off|1Left|2Right|3Both],FellowVehicleLights.Fellow27_VehicleLights.SW_TurnLights[0Off|1Left|2Right|3Both],FellowVehicleLights.Fellow28_VehicleLights.SW_TurnLights[0Off|1Left|2Right|3Both],FellowVehicleLights.Fellow29_VehicleLights.SW_TurnLights[0Off|1Left|2Right|3Both],FellowVehicleLights.Fellow30_VehicleLights.SW_TurnLights[0Off|1Left|2Right|3Both]
  Cast_to_boolean : DataTypeConversion  OutDataTypeStr=boolean  SaturateOnIntegerOverflow=off  RndMeth=Floor
  Cast_to_uint32 : DataTypeConversion  OutDataTypeStr=uint32  SaturateOnIntegerOverflow=off  RndMeth=Floor
  Cast_to_uint32_ : DataTypeConversion  OutDataTypeStr=uint32  SaturateOnIntegerOverflow=off  RndMeth=Floor
  Mux : Mux  Inputs=30
  Mux1 : Mux  Inputs=30
  Mux2 : Mux  Inputs=30
  SW_ManualControl_Lights[1Scheduler|2Manual] : Outport
  SW_BrakeLight[0Off|1On] : Outport  Port=2
  SW_TurnLight[0Off|1Left|2Right|3Both] : Outport  Port=3
  wires:
  Bus Selector3/30 -> Mux2/30  "<SW_TurnLights[0Off|1Left|2Right|3Both]>"
  Bus Selector3/29 -> Mux2/29  "<SW_TurnLights[0Off|1Left|2Right|3Both]>"
  Bus Selector3/28 -> Mux2/28  "<SW_TurnLights[0Off|1Left|2Right|3Both]>"
  Bus Selector3/27 -> Mux2/27  "<SW_TurnLights[0Off|1Left|2Right|3Both]>"
  Bus Selector3/26 -> Mux2/26  "<SW_TurnLights[0Off|1Left|2Right|3Both]>"
  Bus Selector3/25 -> Mux2/25  "<SW_TurnLights[0Off|1Left|2Right|3Both]>"
  Bus Selector3/24 -> Mux2/24  "<SW_TurnLights[0Off|1Left|2Right|3Both]>"
  Bus Selector3/23 -> Mux2/23  "<SW_TurnLights[0Off|1Left|2Right|3Both]>"
  Bus Selector3/22 -> Mux2/22  "<SW_TurnLights[0Off|1Left|2Right|3Both]>"
  Bus Selector3/21 -> Mux2/21  "<SW_TurnLights[0Off|1Left|2Right|3Both]>"
  Bus Selector3/20 -> Mux2/20  "<SW_TurnLights[0Off|1Left|2Right|3Both]>"
  Bus Selector3/19 -> Mux2/19  "<SW_TurnLights[0Off|1Left|2Right|3Both]>"
  Bus Selector3/18 -> Mux2/18  "<SW_TurnLights[0Off|1Left|2Right|3Both]>"
  Bus Selector3/17 -> Mux2/17  "<SW_TurnLights[0Off|1Left|2Right|3Both]>"
  Bus Selector3/16 -> Mux2/16  "<SW_TurnLights[0Off|1Left|2Right|3Both]>"
  Bus Selector3/15 -> Mux2/15  "<SW_TurnLights[0Off|1Left|2Right|3Both]>"
  Bus Selector3/14 -> Mux2/14  "<SW_TurnLights[0Off|1Left|2Right|3Both]>"
  Bus Selector3/13 -> Mux2/13  "<SW_TurnLights[0Off|1Left|2Right|3Both]>"
  Bus Selector3/12 -> Mux2/12  "<SW_TurnLights[0Off|1Left|2Right|3Both]>"
  Bus Selector3/11 -> Mux2/11  "<SW_TurnLights[0Off|1Left|2Right|3Both]>"
  Bus Selector3/10 -> Mux2/10  "<SW_TurnLights[0Off|1Left|2Right|3Both]>"
  Bus Selector3/9 -> Mux2/9  "<SW_TurnLights[0Off|1Left|2Right|3Both]>"
  Bus Selector3/8 -> Mux2/8  "<SW_TurnLights[0Off|1Left|2Right|3Both]>"
  Bus Selector3/7 -> Mux2/7  "<SW_TurnLights[0Off|1Left|2Right|3Both]>"
  Bus Selector3/6 -> Mux2/6  "<SW_TurnLights[0Off|1Left|2Right|3Both]>"
  Bus Selector3/5 -> Mux2/5  "<SW_TurnLights[0Off|1Left|2Right|3Both]>"
  Bus Selector3/4 -> Mux2/4  "<SW_TurnLights[0Off|1Left|2Right|3Both]>"
  Bus Selector3/3 -> Mux2/3  "<SW_TurnLights[0Off|1Left|2Right|3Both]>"
  Bus Selector3/2 -> Mux2/2  "<SW_TurnLights[0Off|1Left|2Right|3Both]>"
  Bus Selector3/1 -> Mux2/1  "<SW_TurnLights[0Off|1Left|2Right|3Both]>"
  Bus Selector2/30 -> Mux1/30  "<SW_BrakeLight[0Off|1On]>"
  Bus Selector2/29 -> Mux1/29  "<SW_BrakeLight[0Off|1On]>"
  Bus Selector2/28 -> Mux1/28  "<SW_BrakeLight[0Off|1On]>"
  Bus Selector2/27 -> Mux1/27  "<SW_BrakeLight[0Off|1On]>"
  Bus Selector2/26 -> Mux1/26  "<SW_BrakeLight[0Off|1On]>"
  Bus Selector2/25 -> Mux1/25  "<SW_BrakeLight[0Off|1On]>"
  Bus Selector2/24 -> Mux1/24  "<SW_BrakeLight[0Off|1On]>"
  Bus Selector2/23 -> Mux1/23  "<SW_BrakeLight[0Off|1On]>"
  Bus Selector2/22 -> Mux1/22  "<SW_BrakeLight[0Off|1On]>"
  Bus Selector2/21 -> Mux1/21  "<SW_BrakeLight[0Off|1On]>"
  Bus Selector2/20 -> Mux1/20  "<SW_BrakeLight[0Off|1On]>"
  Bus Selector2/19 -> Mux1/19  "<SW_BrakeLight[0Off|1On]>"
  Bus Selector2/18 -> Mux1/18  "<SW_BrakeLight[0Off|1On]>"
  Bus Selector2/17 -> Mux1/17  "<SW_BrakeLight[0Off|1On]>"
  Bus Selector2/16 -> Mux1/16  "<SW_BrakeLight[0Off|1On]>"
  Bus Selector2/15 -> Mux1/15  "<SW_BrakeLight[0Off|1On]>"
  Bus Selector2/14 -> Mux1/14  "<SW_BrakeLight[0Off|1On]>"
  Bus Selector2/13 -> Mux1/13  "<SW_BrakeLight[0Off|1On]>"
  Bus Selector2/12 -> Mux1/12  "<SW_BrakeLight[0Off|1On]>"
  Bus Selector2/11 -> Mux1/11  "<SW_BrakeLight[0Off|1On]>"
  Bus Selector2/10 -> Mux1/10  "<SW_BrakeLight[0Off|1On]>"
  Bus Selector2/9 -> Mux1/9  "<SW_BrakeLight[0Off|1On]>"
  Bus Selector2/8 -> Mux1/8  "<SW_BrakeLight[0Off|1On]>"
  Bus Selector2/7 -> Mux1/7  "<SW_BrakeLight[0Off|1On]>"
  Bus Selector2/6 -> Mux1/6  "<SW_BrakeLight[0Off|1On]>"
  Bus Selector2/5 -> Mux1/5  "<SW_BrakeLight[0Off|1On]>"
  Bus Selector2/4 -> Mux1/4  "<SW_BrakeLight[0Off|1On]>"
  Bus Selector2/3 -> Mux1/3  "<SW_BrakeLight[0Off|1On]>"
  Bus Selector2/2 -> Mux1/2  "<SW_BrakeLight[0Off|1On]>"
  Bus Selector2/1 -> Mux1/1  "<SW_BrakeLight[0Off|1On]>"
  Mux2/1 -> Cast_to_uint32_/1
  Mux1/1 -> Cast_to_boolean/1
  Bus Selector1/30 -> Mux/30  "<SW_ManualControl_Lights[1Scheduler|2Manual]>"
  Bus Selector1/29 -> Mux/29  "<SW_ManualControl_Lights[1Scheduler|2Manual]>"
  Bus Selector1/28 -> Mux/28  "<SW_ManualControl_Lights[1Scheduler|2Manual]>"
  Bus Selector1/27 -> Mux/27  "<SW_ManualControl_Lights[1Scheduler|2Manual]>"
  Bus Selector1/26 -> Mux/26  "<SW_ManualControl_Lights[1Scheduler|2Manual]>"
  Bus Selector1/25 -> Mux/25  "<SW_ManualControl_Lights[1Scheduler|2Manual]>"
  Bus Selector1/24 -> Mux/24  "<SW_ManualControl_Lights[1Scheduler|2Manual]>"
  Bus Selector1/23 -> Mux/23  "<SW_ManualControl_Lights[1Scheduler|2Manual]>"
  Bus Selector1/22 -> Mux/22  "<SW_ManualControl_Lights[1Scheduler|2Manual]>"
  Bus Selector1/21 -> Mux/21  "<SW_ManualControl_Lights[1Scheduler|2Manual]>"
  Bus Selector1/20 -> Mux/20  "<SW_ManualControl_Lights[1Scheduler|2Manual]>"
  Bus Selector1/19 -> Mux/19  "<SW_ManualControl_Lights[1Scheduler|2Manual]>"
  Bus Selector1/18 -> Mux/18  "<SW_ManualControl_Lights[1Scheduler|2Manual]>"
  Bus Selector1/17 -> Mux/17  "<SW_ManualControl_Lights[1Scheduler|2Manual]>"
  Bus Selector1/16 -> Mux/16  "<SW_ManualControl_Lights[1Scheduler|2Manual]>"
  Bus Selector1/15 -> Mux/15  "<SW_ManualControl_Lights[1Scheduler|2Manual]>"
  Bus Selector1/14 -> Mux/14  "<SW_ManualControl_Lights[1Scheduler|2Manual]>"
  Bus Selector1/13 -> Mux/13  "<SW_ManualControl_Lights[1Scheduler|2Manual]>"
  Bus Selector1/12 -> Mux/12  "<SW_ManualControl_Lights[1Scheduler|2Manual]>"
  Bus Selector1/11 -> Mux/11  "<SW_ManualControl_Lights[1Scheduler|2Manual]>"
  Bus Selector1/10 -> Mux/10  "<SW_ManualControl_Lights[1Scheduler|2Manual]>"
  Bus Selector1/9 -> Mux/9  "<SW_ManualControl_Lights[1Scheduler|2Manual]>"
  Bus Selector1/8 -> Mux/8  "<SW_ManualControl_Lights[1Scheduler|2Manual]>"
  Bus Selector1/7 -> Mux/7  "<SW_ManualControl_Lights[1Scheduler|2Manual]>"
  Bus Selector1/6 -> Mux/6  "<SW_ManualControl_Lights[1Scheduler|2Manual]>"
  Bus Selector1/5 -> Mux/5  "<SW_ManualControl_Lights[1Scheduler|2Manual]>"
  Bus Selector1/4 -> Mux/4  "<SW_ManualControl_Lights[1Scheduler|2Manual]>"
  Bus Selector1/3 -> Mux/3  "<SW_ManualControl_Lights[1Scheduler|2Manual]>"
  Bus Selector1/2 -> Mux/2  "<SW_ManualControl_Lights[1Scheduler|2Manual]>"
  Bus Selector1/1 -> Mux/1  "<SW_ManualControl_Lights[1Scheduler|2Manual]>"
  Mux/1 -> Cast_to_uint32/1
  Cast_to_boolean/1 -> SW_BrakeLight[0Off|1On]/1
  Fellow_VehicleLights/1 -> Bus Selector1/1, Bus Selector2/1, Bus Selector3/1
  Cast_to_uint32/1 -> SW_ManualControl_Lights[1Scheduler|2Manual]/1
  Cast_to_uint32_/1 -> SW_TurnLight[0Off|1Left|2Right|3Both]/1

== system ASM_Traffic/AnimationInterface/Vehicle_Lights/Coding ==
  In : Inport
  BitwiseOR : simulink/Logic and Bit Operations/Bitwise Operator  logicop=OR  UseBitMask=off  NumInputPorts=3  BitMask=bin2dec('11011001')  BitMaskRealWorld=Stored Integer
  CastToInteger : DataTypeConversion  OutDataTypeStr=uint32  SaturateOnIntegerOverflow=off  RndMeth=Floor
  CastToInteger1 : DataTypeConversion  OutDataTypeStr=uint32  SaturateOnIntegerOverflow=off  RndMeth=Floor
  Demux : Demux  Outputs=3
  Gain : Gain  Gain=15  ParamDataTypeStr=uint32  OutDataTypeStr=uint32
  Gain1 : Gain  Gain=15  ParamDataTypeStr=uint32  OutDataTypeStr=uint32
  Gain2 : Gain  Gain=15  ParamDataTypeStr=uint32  OutDataTypeStr=uint32
  Shift Arithmetic : ArithShift  BitShiftNumber=4  BitShiftDirection=Left
  Shift Arithmetic1 : ArithShift  BitShiftNumber=8  BitShiftDirection=Left
  SwitchDelay : Subsystem
  Out : Outport  VectorParamsAs1DForOutWhenUnconnected=off
  wires:
  SwitchDelay/2(Turnlight_R_out) -> Gain2/1
  SwitchDelay/1(Turnlight_L_out) -> Gain1/1
  Demux/3 -> SwitchDelay/2(Turnlight_R)
  Demux/2 -> SwitchDelay/1(Turnlight_L)
  In/1 -> CastToInteger/1
  Gain/1 -> BitwiseOR/1
  Gain1/1 -> Shift Arithmetic/1
  Gain2/1 -> Shift Arithmetic1/1
  Shift Arithmetic/1 -> BitwiseOR/2
  Shift Arithmetic1/1 -> BitwiseOR/3
  CastToInteger/1 -> Demux/1
  Demux/1 -> Gain/1
  BitwiseOR/1 -> CastToInteger1/1
  CastToInteger1/1 -> Out/1

== system ASM_Traffic/DomainControl/DriverAssistance/Control ==
  note: Driver Assistance
  Interface_In : Inport
  Bus Creator : BusCreator  Inputs=2
  SoftECU_ACC : Subsystem
  Sw_ECU_Signals : Subsystem
  UserInterface : Subsystem
  Control : Outport  VectorParamsAs1DForOutWhenUnconnected=off
  wires:
  Bus Creator/1 -> Control/1  "Control"
  Sw_ECU_Signals/1(ECU_Signals) -> Bus Creator/2
  SoftECU_ACC/2(Out) -> Sw_ECU_Signals/1(SoftECU)
  Interface_In/1 -> Sw_ECU_Signals/2(ExternalECU), SoftECU_ACC/2(Interface_In), UserInterface/1(Interface_In)
  SoftECU_ACC/1(ASMSignalBus) -> Bus Creator/1, UserInterface/2(In)
  UserInterface/1(Out) -> SoftECU_ACC/1(UserInterface)
